simulink model "solar_pv_protected_c07_circuit"  (R2026b)
settings: Solver=VariableStepAuto
model workspace (MAT data in the model file):
  candidate_owner = 'pv_protection_integration_20261023_r01'
  solar_edit_metadata : object (value not decoded)
libraries: fl_lib x149, ee_lib x16, ltc4364demo_lib x3, batteryecm_lib x1, solarprotect_lib x1
(part 8 of 16)

== system solar_pv_protected_c07_circuit/D3 ==
  Native_Diode : ee_lib/Semiconductors & Converters/Diode  Description=|  Vf=0.6 V  Ron=0.3 Ohm  Goff=1e-8 S  N_series=1  N_parallel=1  ZenerEnable=false  BV=30 V  Rz=0.3 Ohm  enable_fault_composite=simscape.enum.onoff.off  i_specify=off  i_priority=None  i=0 A  i_nominal_specify=off  i_nominal_value=1  i_nominal_unit=A  v_specify=off  v_priority=None  v=0 V  v_nominal_specify=off  v_nominal_value=1  v_nominal_unit=V  ModelType=ee.enum.diode.idealModelType.pwl  TableType=ee.enum.diode.tableType.IfMat  IfMat=[.07, .12, .19, 1.75, 4.24, 7.32, 11.2; .16, .3, .72, 2.14, 5.02, 8.35, 13.12] A  VfMat=[.9, 1.15, 1.25, 1.5, 1.75, 2.17, 2.6, 2.85; .58, .68, .75, 1.1, 1.38, 1.77, 2.27, 2.7] V  TjVec=[25, 125] degC  VfVec=[.5, .7, .9, 1.3, 1.7, 2.1, 2.5] V  IfVec=[.1, .2, .5, 1, 2, 4, 7, 10] A  IrMat=[1e-06, 2e-06, 5e-06, 1e-05, 2.5e-05, 5e-05, .0001; 2e-06, 5e-06, 1e-05, 4e-05, 8e-05, .0002, .0005] A  VrMat=[10, 100, 200, 250, 300, 325, 350; 10, 70, 160, 220, 270, 300, 320] V  VrVec=[10, 20, 40, 50, 70, 80, 100] V  IrVec=[1e-06, 2e-06, 5e-06, 1e-05, 2e-05, 5e-05, .0001] A  rec_loss_model=ee.enum.diode.reverseRecoveryModelTabulateUpTo3D.fixed  ErecVal=0 J  scaleWithIandV=true  ErecMat=zeros(2, 3) J  ErecMat3D=zeros(2, 3, 2) J  TjrecVec=[25, 125] degC  IfrecVec=[.1, 1, 10] A  IrecVal=10 A  VrecVal=10 V  VrecVec=[0, 100] V  tFilter=1 / 1000 / 100 s  thermal_network_parameterization=ee.enum.thermalNetworkTopology.junctionCase  Rth=[0, 10] K/W  Rth_Cauer=[1, 3, 10] K/W  Rth_Foster=[.08, .14, .22, .16] K/W  thermal_mass_parameterization=ee.enum.thermalNetwork.timeconstant  thermal_mass=[0, 1] J/K  thermal_mass_Cauer=[.1, .3, 1] J/K  thermal_mass_Foster=[.001, .005, .05, .5] J/K  thermal_time_constant=[0, 10] s  thermal_time_constant_Cauer=[1, 3, 10] s  thermal_time_constant_Foster=[7e-05, .0007, .01, .08] s  thermal_mass_initial_temperatures=[25, 25] degC  thermal_mass_initial_temperatures_Cauer=[25, 25, 25] degC  thermal_mass_initial_temperatures_Foster=[25, 25, 25, 25] degC  junction_thermal_mass=0.01 J/K  junction_temperature_specify=off  junction_temperature_priority=None  junction_temperature=25 degC  junction_temperature_nominal_specify=off  junction_temperature_nominal_value=1  junction_temperature_nominal_unit=degC  ThermalPort=false  ModelTypePhysical=ee.enum.diode.physicalModelType.exponential  prmExp=ee.enum.diode.expParam.useTwo  I12=[.0137, .545] A  V12=[.6, .7] V  IS=1e-12 A  ec=1  I1=0.0137 A  V1=0.6 V  RS=0 Ohm  C_param=ee.enum.diode.capParam.fixed  CJ=0 pF  CJ0=5 pF  Vvec=[.1, 10, 100] V  Cvec=[3.5, 1, .4] pF  VJ=1 V  Mgrad=0.5  FC=0.5  Q_param=ee.enum.diode.recoveryParam.off  iRM=-7.15 A  iF=4 A  didt=-750 A/us  trr_factor=3  trr=115 ns  Qrr=150 nA*s  Vr=-600 V  Ls=150 nH  Erec=0.03 J  TT=50 ns  tau=100 ns  T_param=ee.enum.diode.temperatureParam.off  Tmeas=25 degC  I1_T2=0.245 A  V1_T2=0.5 V  IS_T2=1.25e-7 A  Tmeas2=125 degC  EG_param=ee.enum.diode.egapParam.material_si  EG=1.11 eV  XTI_param=ee.enum.diode.xtiParam.pn  XTI=3  dBVdT=0 V/K  Tdevice=25 degC  i_capacitor_specify=off  i_capacitor_priority=None  i_capacitor=0 A  i_capacitor_nominal_specify=off  i_capacitor_nominal_value=1  i_capacitor_nominal_unit=A  Qj_specify=off  Qj_priority=None  Qj=0 C  Qj_nominal_specify=off  Qj_nominal_value=1  Qj_nominal_unit=uC
      | この回路での名前　　; D3/Native_Diode（内部モデル）
      | 部品名　　　　　　　; D3 / SS14-E3/61Tの内部表現
      | この回路での役割　　; マイコン電源へ向かうダイオードD3の、順方向と逆方向で異なる電流の流れ方をモデル内部で表す要素。
      | ここでの動き　　　　; 実部品D3の内部表現として標準ダイオードを使う。別のダイオードを追加した意味ではなく、型番固有の全特性を再現しているものでもない。
      | 
      | 【モデルの詳細・確認の範囲】
      | モデル内区分　　　　; 実部品D3の内部数値表現。独立した追加部品ではない。
      | 対応する実部品　　　; D3 / SS14-E3/61T
      | モデルの範囲　　　　; Simscapeダイオード素子による近似。順方向損失、漏れ、温度依存、逆回復・接合容量の型番固有特性を完全に再現するものではない。
      | 説明の参照　　　　　; 上位部品ブロックのDescriptionに目的・接続・型番・未確認事項を記す。
      | 確認の範囲　　　　　; 説明整理のみ。実部品の全特性への同定や新たな動作試験を示さない。
      settings: AttributesFormatString=SS14-E3/61T
  Pin_001 : PMIOPort  Description=|  Side=Left  ConnectionType=Connection: foundation.electrical.electrical
      | 識別名　　　　　　　; Pin_001
      | 種別　　　　　　　　; Simscape Connection Port（階層境界の物理端子）
      | 所属部品　　　　　　; D3
      | 配置目的　　　　　　; 内部の電気ノードを、この外箱の外側の対応端子へ引き出す。
      | 対応端子　　　　　　; lconn:1／2番 A
      | 接続ラベル　　　　　; P5
      | モデルの範囲　　　　; 実部品を1個追加する表現ではない。端子自体に増幅・遮断・測定機能を持たない。
      | 端子番号の注意　　　; Connection Portの番号は外箱内の対応番号であり、実パッケージのピン番号とは区別する。
      | 確認の範囲　　　　　; 実ポートと階層対応による静的接続の説明。電気特性の再現性は所属部品の説明を参照する。
  Pin_002 : PMIOPort  Description=|  Port=2  Side=Right  ConnectionType=Connection: foundation.electrical.electrical
      | 識別名　　　　　　　; Pin_002
      | 種別　　　　　　　　; Simscape Connection Port（階層境界の物理端子）
      | 所属部品　　　　　　; D3
      | 配置目的　　　　　　; 内部の電気ノードを、この外箱の外側の対応端子へ引き出す。
      | 対応端子　　　　　　; rconn:1／1番 K
      | 接続ラベル　　　　　; VSYS_5V
      | モデルの範囲　　　　; 実部品を1個追加する表現ではない。端子自体に増幅・遮断・測定機能を持たない。
      | 端子番号の注意　　　; Connection Portの番号は外箱内の対応番号であり、実パッケージのピン番号とは区別する。
      | 確認の範囲　　　　　; 実ポートと階層対応による静的接続の説明。電気特性の再現性は所属部品の説明を参照する。
  connections:
  Pin_001/RConn1 -- Native_Diode/LConn1
  Pin_002/RConn1 -- Native_Diode/RConn1
